simulink model "simulink_filter"  (R2024a)
settings: Solver=VariableStepAuto  StartTime=0.0  StopTime=30.0  RelTol=1e-3
settings Model: Creator=User  LastModifiedBy=User

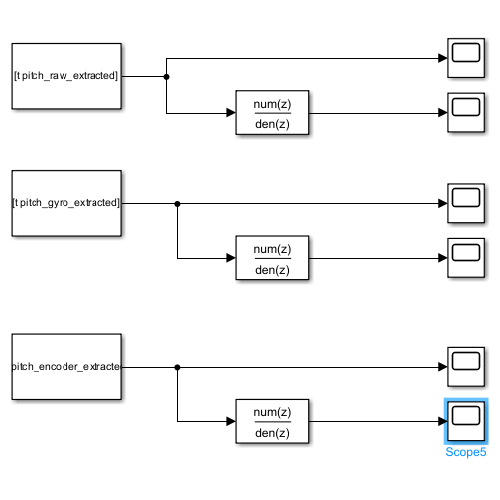
[thumbnail: Simulink's stored preview of the top-level diagram]
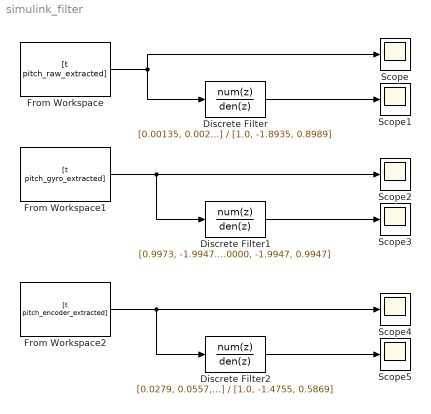
== system simulink_filter ==
  Discrete Filter : DiscreteFilter  Numerator=[0.00135, 0.00270, 0.00135]  Denominator=[1.0, -1.8935, 0.8989]
  Discrete Filter1 : DiscreteFilter  Numerator=[0.9973, -1.9947, 0.9973]  Denominator=[1.0000, -1.9947, 0.9947]
  Discrete Filter2 : DiscreteFilter  Numerator=[0.0279, 0.0557, 0.0279]  Denominator=[1.0, -1.4755, 0.5869]
  From Workspace : FromWorkspace  VariableName=[t pitch_raw_extracted]  SampleTime=0.006  Interpolate=off  OutputAfterFinalValue=Holding final value
  From Workspace1 : FromWorkspace  VariableName=[t pitch_gyro_extracted]  SampleTime=0.006  Interpolate=off  OutputAfterFinalValue=Holding final value
  From Workspace2 : FromWorkspace  VariableName=[t pitch_encoder_extracted]  SampleTime=0.006  Interpolate=off  OutputAfterFinalValue=Holding final value
  Scope{,1..5} (6 alike) : Scope
  wires:
  From Workspace/1 -> Scope/1, Discrete Filter/1
  Discrete Filter/1 -> Scope1/1
  From Workspace1/1 -> Discrete Filter1/1, Scope2/1
  Discrete Filter1/1 -> Scope3/1
  Discrete Filter2/1 -> Scope5/1
  From Workspace2/1 -> Discrete Filter2/1, Scope4/1
